simulink model "Pierre_Controller_LTI_2026b"  (R2025b)
settings: Solver=ode1  StartTime=0.0  StopTime=inf  FixedStep=Ts  RelTol=1e-3
PostLoadFcn:
  | , if any(exist('dsrtsu_mdlpostloadfcn', 'file') ~= 0), dsrtsu_mdlpostloadfcn('Execute', bdroot); end,
InitFcn:
  | , if any(exist('rtifpga_mdlclblib', 'file') ~= 0), rtifpga_mdlclblib('Init', bdroot); end,
values from neighbouring files (symbols this model uses):
  BUTTER = ss(A,B,C,D,Ts)    [build_model.m]
  K = opensave.K_final    [build_model.m]
  Px = 1    [build_model.m]
  Py = 1    [build_model.m]
  Pz = 1    [build_model.m]
  S_Sensor = 0.1134    [build_model.m]
  Sen_AX = 2.0176    [build_model.m]
  Sen_AY = 2.011    [build_model.m]
  Sen_AZ = 2.0066    [build_model.m]
  Sen_GX = 0.75481    [build_model.m]
  Sen_GY = 0.75728    [build_model.m]
  Sen_GZ = 0.74931    [build_model.m]
  Sweep_amp = 0.5    [build_model.m]
  Switch_excit = 4    [build_model.m]
  TMS_amp = 2    [build_model.m]
  TMS_freq1 = 80    [build_model.m]
  TMS_freq2 = 0    [build_model.m]
  TMS_freq3 = 0    [build_model.m]
  Ts = 1/Fs    (= 0.001)    [build_model.m]
  V_sat = 2/10    (= 0.2)    [build_model.m]
  V_sat_TMS = 5    [build_model.m]
undefined symbols (not defined in the file or in its folder): R, S
libraries: dspfdesign x15, rti1202lib_adc_class1 x10, rti1202lib_dac_class1 x7, rti1202lib_adc_class2 x6, dspxfrm3 x3, cstblocks x1, simulink x1
(part 2 of 3)

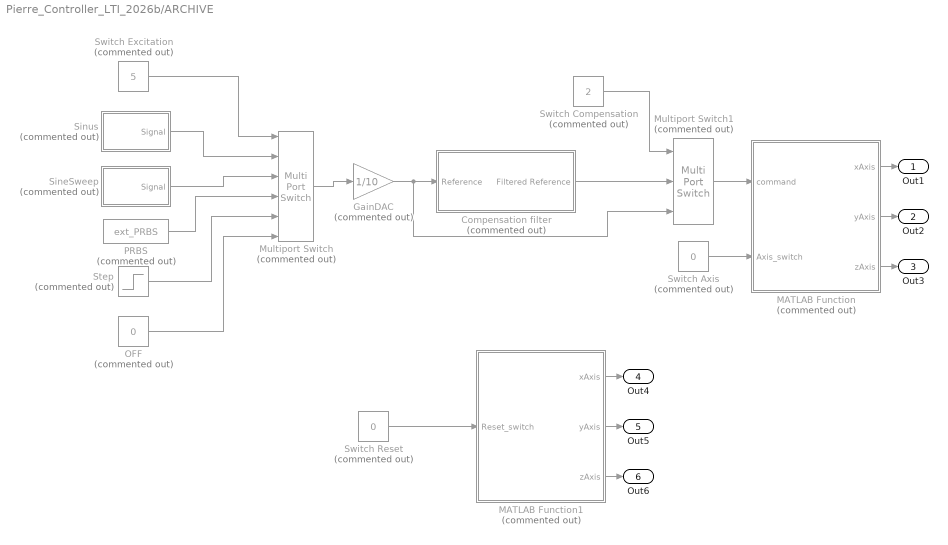
== system Pierre_Controller_LTI_2026b/ARCHIVE ==
  Compensation filter : Subsystem  Commented=on
  GainDAC : Gain  Commented=on  Gain=1/10
  MATLAB Function : MATLAB Function  Commented=on  TreatAsAtomicUnit=on
  MATLAB Function1 : MATLAB Function  Commented=on  TreatAsAtomicUnit=on  SystemSampleTime=Ts
  Multiport Switch : MultiPortSwitch  Commented=on  Inputs=5  DiagnosticForDefault=Warning  SaturateOnIntegerOverflow=off  InputSameDT=off
  Multiport Switch1 : MultiPortSwitch  Commented=on  Inputs=2  DiagnosticForDefault=Warning  SaturateOnIntegerOverflow=off  InputSameDT=off
  OFF : Constant  Commented=on  Value=0
  PRBS : FromWorkspace  Commented=on  VariableName=ext_PRBS  SampleTime=-1
  SineSweep : Subsystem  Commented=on
  Sinus : Subsystem  Commented=on
  Step : Step  Commented=on  Time=5  After=0.5  SampleTime=Ts
  Switch Axis : Constant  Commented=on  Value=0
  Switch Compensation : Constant  Commented=on  Value=2
  Switch Excitation : Constant  Commented=on  Value=5
  Switch Reset : Constant  Commented=on  Value=0  SampleTime=Ts
  Out1 : Outport  VectorParamsAs1DForOutWhenUnconnected=off
  Out2 : Outport  Port=2  VectorParamsAs1DForOutWhenUnconnected=off
  Out3 : Outport  Port=3  VectorParamsAs1DForOutWhenUnconnected=off
  Out4 : Outport  Port=4  VectorParamsAs1DForOutWhenUnconnected=off
  Out5 : Outport  Port=5  VectorParamsAs1DForOutWhenUnconnected=off
  Out6 : Outport  Port=6  VectorParamsAs1DForOutWhenUnconnected=off
  wires:
  PRBS/1 -> Multiport Switch/4
  Switch Axis/1 -> MATLAB Function/2(Axis_switch)
  SineSweep/1(Signal) -> Multiport Switch/3
  Multiport Switch/1 -> GainDAC/1
  Sinus/1(Signal) -> Multiport Switch/2
  Switch Excitation/1 -> Multiport Switch/1
  Switch Compensation/1 -> Multiport Switch1/1
  GainDAC/1 -> Multiport Switch1/3, Compensation filter/1(Reference)
  Compensation filter/1(Filtered Reference) -> Multiport Switch1/2
  OFF/1 -> Multiport Switch/6
  Multiport Switch1/1 -> MATLAB Function/1(command)
  Step/1 -> Multiport Switch/5
  Switch Reset/1 -> MATLAB Function1/1(Reset_switch)
  MATLAB Function1/2(yAxis) -> Out5/1
  MATLAB Function/2(yAxis) -> Out2/1
  MATLAB Function1/1(xAxis) -> Out4/1
  MATLAB Function1/3(zAxis) -> Out6/1
  MATLAB Function/1(xAxis) -> Out1/1
  MATLAB Function/3(zAxis) -> Out3/1

== system Pierre_Controller_LTI_2026b/Clock ==
  Clock : Clock
  Timestamp : Outport  VectorParamsAs1DForOutWhenUnconnected=off
  wires:
  Clock/1 -> Timestamp/1

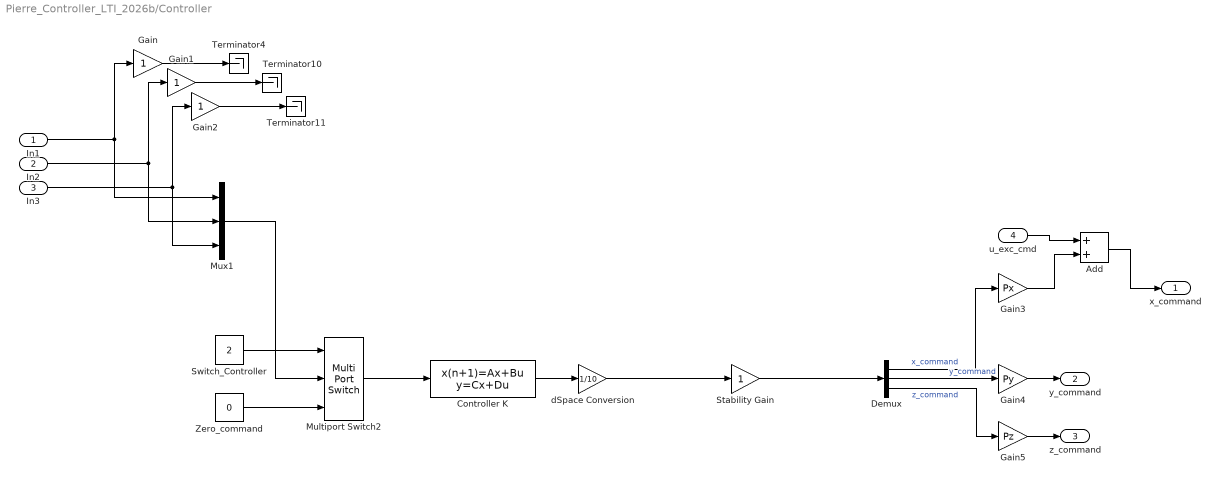
== system Pierre_Controller_LTI_2026b/Controller ==
  In1 : Inport
  In2 : Inport  Port=2
  In3 : Inport  Port=3
  u_exc_cmd : Inport  Port=4
  Add : Sum
  Controller K : DiscreteStateSpace  A=K.A  B=K.B  C=K.C  D=K.D  SampleTime=-1
  Demux : Demux  Outputs=3
  Gain : Gain
  Gain1 : Gain
  Gain2 : Gain
  Gain3 : Gain  Gain=Px
  Gain4 : Gain  Gain=Py
  Gain5 : Gain  Gain=Pz
  Multiport Switch2 : MultiPortSwitch  Inputs=2  DiagnosticForDefault=None  SaturateOnIntegerOverflow=off  InputSameDT=off
  Mux1 : Mux  Inputs=3
  Stability Gain : Gain
  Switch_Controller : Constant  Value=2
  Terminator10 : Terminator
  Terminator11 : Terminator
  Terminator4 : Terminator
  Zero_command : Constant  Value=0  VectorParams1D=off
  dSpace Conversion : Gain  Gain=1/10
  x_command : Outport  VectorParamsAs1DForOutWhenUnconnected=off
  y_command : Outport  Port=2  VectorParamsAs1DForOutWhenUnconnected=off
  z_command : Outport  Port=3  VectorParamsAs1DForOutWhenUnconnected=off
  wires:
  Switch_Controller/1 -> Multiport Switch2/1
  Mux1/1 -> Multiport Switch2/2
  Zero_command/1 -> Multiport Switch2/3
  Demux/2 -> Gain4/1  "y_command"
  Demux/3 -> Gain5/1  "z_command"
  Demux/1 -> Gain3/1  "x_command"
  In2/1 -> Mux1/2, Gain1/1
  In1/1 -> Mux1/1, Gain/1
  In3/1 -> Mux1/3, Gain2/1
  Gain2/1 -> Terminator11/1
  Gain1/1 -> Terminator10/1
  Gain/1 -> Terminator4/1
  Controller K/1 -> dSpace Conversion/1
  dSpace Conversion/1 -> Stability Gain/1
  Multiport Switch2/1 -> Controller K/1
  Gain3/1 -> Add/2
  Gain4/1 -> y_command/1
  Gain5/1 -> z_command/1
  Stability Gain/1 -> Demux/1
  Add/1 -> x_command/1
  u_exc_cmd/1 -> Add/1

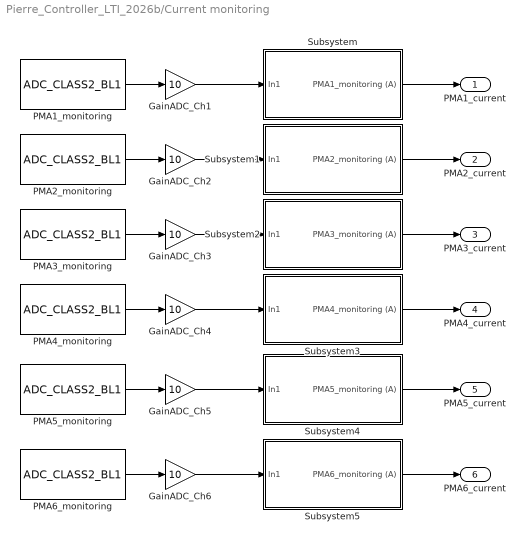
== system Pierre_Controller_LTI_2026b/Current monitoring ==
  GainADC_Ch{1..6} (6 alike) : Gain  Gain=10
  PMA1_monitoring : rti1202lib_adc_class2/ADC_CLASS2_BL1  DSProperties=struct('RTI',struct('Version',uint32(1),'BlockType',struct('isSLSource',uint8(1),'isSLSink',uint8(1),'isHWSource',uint8(0),'isHWSink',uint8(1),'isSetup',uint8(0),'isInline',uint8(1),'isNonInline',uint8(0),'isInterrupt',uint8(0),'isChannelwise',uint8(1)),'IOBoardType',{{'DS120X','STD','ADCC2'}},'UnitType','ADC','Identifier','ADC','DialogType','ML','BlockSet','NONE','SlaveProcessor','NONE'))  RTIBlockInterface=struct('OutputPortsActive',1,'OutputPortsWidth',int32(1),'OutputPortsDataType',{{'SS_DOUBLE'}},'OutputPortsName',{{'ADC'}},'DialogFcn','rti120xstdadcc2adcgui','InitLevel',3,'IconTransparency','on','BlockDisplay',{{['ADC CL2\nChannel: 1'],'center'}},'BlockName',struct('Token',{{'ADC_CLASS2_BL1'}}))  RTIBlockParameters=struct('ChannelNo',{{1,'OFF',[]}},'TLCFileName',{{'rti120xadc_c2_adc','OFF',[]}})  RTISFcnParameters=struct('ChannelNo','int16','TLCFileName','char')  RTIBlockParaDefault=struct('ChannelNo',1,'TLCFileName','rti120xadc_c2_adc')
  PMA2_monitoring : rti1202lib_adc_class2/ADC_CLASS2_BL1  DSProperties=struct('RTI',struct('Version',uint32(1),'BlockType',struct('isSLSource',uint8(1),'isSLSink',uint8(1),'isHWSource',uint8(0),'isHWSink',uint8(1),'isSetup',uint8(0),'isInline',uint8(1),'isNonInline',uint8(0),'isInterrupt',uint8(0),'isChannelwise',uint8(1)),'IOBoardType',{{'DS120X','STD','ADCC2'}},'UnitType','ADC','Identifier','ADC','DialogType','ML','BlockSet','NONE','SlaveProcessor','NONE'))  RTIBlockInterface=struct('OutputPortsActive',1,'OutputPortsWidth',int32(1),'OutputPortsDataType',{{'SS_DOUBLE'}},'OutputPortsName',{{'ADC'}},'DialogFcn','rti120xstdadcc2adcgui','InitLevel',3,'IconTransparency','on','BlockDisplay',{{['ADC CL2\nChannel: 2'],'center'}},'BlockName',struct('Token',{{'ADC_CLASS2_BL1'}}))  RTIBlockParameters=struct('ChannelNo',{{2,'OFF',[]}},'TLCFileName',{{'rti120xadc_c2_adc','OFF',[]}})  RTISFcnParameters=struct('ChannelNo','int16','TLCFileName','char')  RTIBlockParaDefault=struct('ChannelNo',1,'TLCFileName','rti120xadc_c2_adc')
  PMA3_monitoring : rti1202lib_adc_class2/ADC_CLASS2_BL1  DSProperties=struct('RTI',struct('Version',uint32(1),'BlockType',struct('isSLSource',uint8(1),'isSLSink',uint8(1),'isHWSource',uint8(0),'isHWSink',uint8(1),'isSetup',uint8(0),'isInline',uint8(1),'isNonInline',uint8(0),'isInterrupt',uint8(0),'isChannelwise',uint8(1)),'IOBoardType',{{'DS120X','STD','ADCC2'}},'UnitType','ADC','Identifier','ADC','DialogType','ML','BlockSet','NONE','SlaveProcessor','NONE'))  RTIBlockInterface=struct('OutputPortsActive',1,'OutputPortsWidth',int32(1),'OutputPortsDataType',{{'SS_DOUBLE'}},'OutputPortsName',{{'ADC'}},'DialogFcn','rti120xstdadcc2adcgui','InitLevel',3,'IconTransparency','on','BlockDisplay',{{['ADC CL2\nChannel: 3'],'center'}},'BlockName',struct('Token',{{'ADC_CLASS2_BL1'}}))  RTIBlockParameters=struct('ChannelNo',{{3,'OFF',[]}},'TLCFileName',{{'rti120xadc_c2_adc','OFF',[]}})  RTISFcnParameters=struct('ChannelNo','int16','TLCFileName','char')  RTIBlockParaDefault=struct('ChannelNo',1,'TLCFileName','rti120xadc_c2_adc')
  PMA4_monitoring : rti1202lib_adc_class2/ADC_CLASS2_BL1  DSProperties=struct('RTI',struct('Version',uint32(1),'BlockType',struct('isSLSource',uint8(1),'isSLSink',uint8(1),'isHWSource',uint8(0),'isHWSink',uint8(1),'isSetup',uint8(0),'isInline',uint8(1),'isNonInline',uint8(0),'isInterrupt',uint8(0),'isChannelwise',uint8(1)),'IOBoardType',{{'DS120X','STD','ADCC2'}},'UnitType','ADC','Identifier','ADC','DialogType','ML','BlockSet','NONE','SlaveProcessor','NONE'))  RTIBlockInterface=struct('OutputPortsActive',1,'OutputPortsWidth',int32(1),'OutputPortsDataType',{{'SS_DOUBLE'}},'OutputPortsName',{{'ADC'}},'DialogFcn','rti120xstdadcc2adcgui','InitLevel',3,'IconTransparency','on','BlockDisplay',{{['ADC CL2\nChannel: 4'],'center'}},'BlockName',struct('Token',{{'ADC_CLASS2_BL1'}}))  RTIBlockParameters=struct('ChannelNo',{{4,'OFF',[]}},'TLCFileName',{{'rti120xadc_c2_adc','OFF',[]}})  RTISFcnParameters=struct('ChannelNo','int16','TLCFileName','char')  RTIBlockParaDefault=struct('ChannelNo',1,'TLCFileName','rti120xadc_c2_adc')
  PMA5_monitoring : rti1202lib_adc_class2/ADC_CLASS2_BL1  DSProperties=struct('RTI',struct('Version',uint32(1),'BlockType',struct('isSLSource',uint8(1),'isSLSink',uint8(1),'isHWSource',uint8(0),'isHWSink',uint8(1),'isSetup',uint8(0),'isInline',uint8(1),'isNonInline',uint8(0),'isInterrupt',uint8(0),'isChannelwise',uint8(1)),'IOBoardType',{{'DS120X','STD','ADCC2'}},'UnitType','ADC','Identifier','ADC','DialogType','ML','BlockSet','NONE','SlaveProcessor','NONE'))  RTIBlockInterface=struct('OutputPortsActive',1,'OutputPortsWidth',int32(1),'OutputPortsDataType',{{'SS_DOUBLE'}},'OutputPortsName',{{'ADC'}},'DialogFcn','rti120xstdadcc2adcgui','InitLevel',3,'IconTransparency','on','BlockDisplay',{{['ADC CL2\nChannel: 5'],'center'}},'BlockName',struct('Token',{{'ADC_CLASS2_BL1'}}))  RTIBlockParameters=struct('ChannelNo',{{5,'OFF',[]}},'TLCFileName',{{'rti120xadc_c2_adc','OFF',[]}})  RTISFcnParameters=struct('ChannelNo','int16','TLCFileName','char')  RTIBlockParaDefault=struct('ChannelNo',1,'TLCFileName','rti120xadc_c2_adc')
  PMA6_monitoring : rti1202lib_adc_class2/ADC_CLASS2_BL1  DSProperties=struct('RTI',struct('Version',uint32(1),'BlockType',struct('isSLSource',uint8(1),'isSLSink',uint8(1),'isHWSource',uint8(0),'isHWSink',uint8(1),'isSetup',uint8(0),'isInline',uint8(1),'isNonInline',uint8(0),'isInterrupt',uint8(0),'isChannelwise',uint8(1)),'IOBoardType',{{'DS120X','STD','ADCC2'}},'UnitType','ADC','Identifier','ADC','DialogType','ML','BlockSet','NONE','SlaveProcessor','NONE'))  RTIBlockInterface=struct('OutputPortsActive',1,'OutputPortsWidth',int32(1),'OutputPortsDataType',{{'SS_DOUBLE'}},'OutputPortsName',{{'ADC'}},'DialogFcn','rti120xstdadcc2adcgui','InitLevel',3,'IconTransparency','on','BlockDisplay',{{['ADC CL2\nChannel: 6'],'center'}},'BlockName',struct('Token',{{'ADC_CLASS2_BL1'}}))  RTIBlockParameters=struct('ChannelNo',{{6,'OFF',[]}},'TLCFileName',{{'rti120xadc_c2_adc','OFF',[]}})  RTISFcnParameters=struct('ChannelNo','int16','TLCFileName','char')  RTIBlockParaDefault=struct('ChannelNo',1,'TLCFileName','rti120xadc_c2_adc')
  Subsystem : Subsystem
  Subsystem1 : Subsystem
  Subsystem2 : Subsystem
  Subsystem3 : Subsystem
  Subsystem4 : Subsystem
  Subsystem5 : Subsystem
  PMA1_current : Outport  VectorParamsAs1DForOutWhenUnconnected=off
  PMA2_current : Outport  Port=2  VectorParamsAs1DForOutWhenUnconnected=off
  PMA3_current : Outport  Port=3  VectorParamsAs1DForOutWhenUnconnected=off
  PMA4_current : Outport  Port=4  VectorParamsAs1DForOutWhenUnconnected=off
  PMA5_current : Outport  Port=5  VectorParamsAs1DForOutWhenUnconnected=off
  PMA6_current : Outport  Port=6  VectorParamsAs1DForOutWhenUnconnected=off
  wires:
  GainADC_Ch6/1 -> Subsystem5/1(In1)
  PMA5_monitoring/1 -> GainADC_Ch5/1
  PMA6_monitoring/1 -> GainADC_Ch6/1
  GainADC_Ch5/1 -> Subsystem4/1(In1)
  GainADC_Ch1/1 -> Subsystem/1(In1)
  PMA1_monitoring/1 -> GainADC_Ch1/1
  PMA2_monitoring/1 -> GainADC_Ch2/1
  GainADC_Ch2/1 -> Subsystem1/1(In1)
  PMA3_monitoring/1 -> GainADC_Ch3/1
  GainADC_Ch3/1 -> Subsystem2/1(In1)
  GainADC_Ch4/1 -> Subsystem3/1(In1)
  PMA4_monitoring/1 -> GainADC_Ch4/1
  Subsystem/1(PMA1_monitoring (A)) -> PMA1_current/1
  Subsystem1/1(PMA2_monitoring (A)) -> PMA2_current/1
  Subsystem2/1(PMA3_monitoring (A)) -> PMA3_current/1
  Subsystem3/1(PMA4_monitoring (A)) -> PMA4_current/1
  Subsystem4/1(PMA5_monitoring (A)) -> PMA5_current/1
  Subsystem5/1(PMA6_monitoring (A)) -> PMA6_current/1

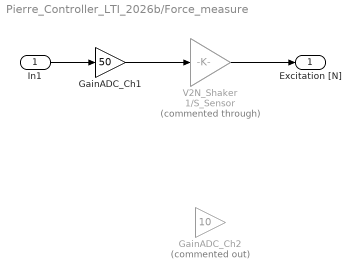
== system Pierre_Controller_LTI_2026b/Force_measure ==
  In1 : Inport
  GainADC_Ch1 : Gain  Gain=50
  GainADC_Ch2 : Gain  Commented=on  Gain=10
  V2N_Shaker : Gain  Commented=through  Gain=1/S_Sensor
  Excitation [N] : Outport  VectorParamsAs1DForOutWhenUnconnected=off
  wires:
  In1/1 -> GainADC_Ch1/1
  V2N_Shaker/1 -> Excitation [N]/1
  GainADC_Ch1/1 -> V2N_Shaker/1

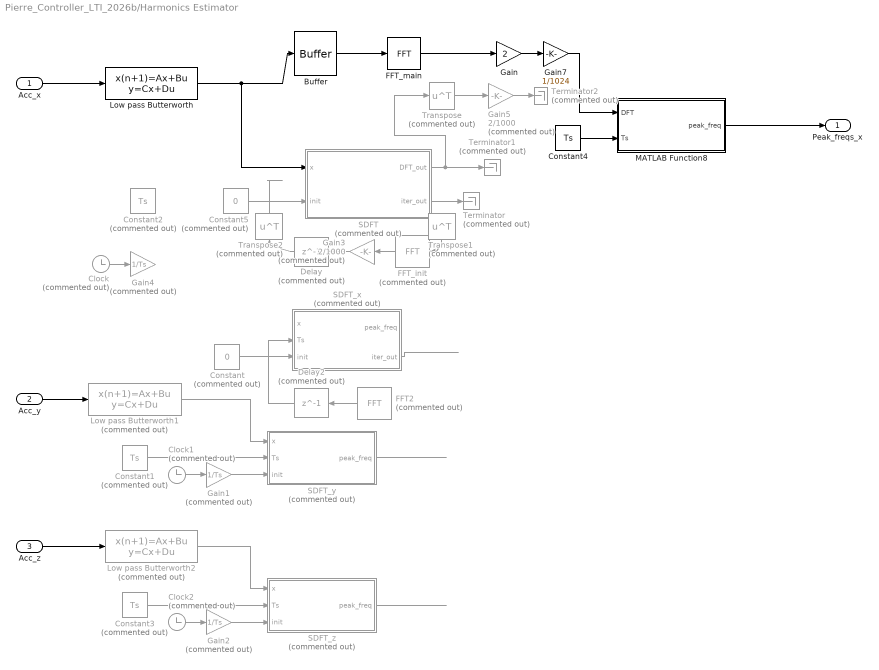
== system Pierre_Controller_LTI_2026b/Harmonics Estimator ==
  Acc_x : Inport
  Acc_y : Inport  Port=2
  Acc_z : Inport  Port=3
  Buffer : Buffer  N=1024  OutputFrames=off
  Clock : Clock  Commented=on
  Clock1 : Clock  Commented=on
  Clock2 : Clock  Commented=on
  Constant : Constant  Commented=on  Value=0
  Constant1 : Constant  Commented=on  Value=Ts  SampleTime=-1
  Constant2 : Constant  Commented=on  Value=Ts  SampleTime=-1
  Constant3 : Constant  Commented=on  Value=Ts  SampleTime=-1
  Constant4 : Constant  Value=Ts  SampleTime=-1
  Constant5 : Constant  Commented=on  Value=0  SampleTime=-1
  Delay : Delay  Commented=on  DelayLength=1  InitialCondition=0
  Delay2 : Delay  Commented=on  DelayLength=1  InitialCondition=0
  FFT2 : dspxfrm3/FFT  Commented=on  FFTImplementation=Auto  CompMethod=Table lookup  TableOpt=NEW  TableOptActive=Speed  BitRevOrder=off  Normalize=off  InheritFFTLength=on  FFTLength=64  WrapInput=on  roundingMode=Floor  overflowMode=off  firstCoeffDataTypeStr=Inherit: Same word length as input  firstCoeffLastDataTypeStr=Inherit: Same word length as input  outputMin=[]  outputMax=[]
  FFT_init : dspxfrm3/FFT  Commented=on  FFTImplementation=Auto  CompMethod=Table lookup  TableOpt=NEW  TableOptActive=Speed  BitRevOrder=off  Normalize=off  InheritFFTLength=on  FFTLength=64  WrapInput=on  roundingMode=Floor  overflowMode=off  firstCoeffDataTypeStr=Inherit: Same word length as input  firstCoeffLastDataTypeStr=Inherit: Same word length as input  outputMin=[]  outputMax=[]
  FFT_main : dspxfrm3/FFT  FFTImplementation=Auto  CompMethod=Table lookup  TableOpt=NEW  TableOptActive=Speed  BitRevOrder=off  Normalize=off  InheritFFTLength=on  FFTLength=64  WrapInput=on  roundingMode=Floor  overflowMode=off  firstCoeffDataTypeStr=Inherit: Same word length as input  firstCoeffLastDataTypeStr=Inherit: Same word length as input  outputMin=[]  outputMax=[]
  Gain : Gain  Gain=2
  Gain1 : Gain  Commented=on  Gain=1/Ts
  Gain2 : Gain  Commented=on  Gain=1/Ts
  Gain3 : Gain  Commented=on  Gain=2/1000
  Gain4 : Gain  Commented=on  Gain=1/Ts
  Gain5 : Gain  Commented=on  Gain=2/1000
  Gain7 : Gain  Gain=1/1024
  Low pass Butterworth : DiscreteStateSpace  A=BUTTER.A  B=BUTTER.B  C=BUTTER.C  D=BUTTER.D  SampleTime=-1
  Low pass Butterworth1 : DiscreteStateSpace  Commented=on  A=BUTTER.A  B=BUTTER.B  C=BUTTER.C  D=BUTTER.D  SampleTime=-1
  Low pass Butterworth2 : DiscreteStateSpace  Commented=on  A=BUTTER.A  B=BUTTER.B  C=BUTTER.C  D=BUTTER.D  SampleTime=-1
  MATLAB Function8 : MATLAB Function  TreatAsAtomicUnit=on
  SDFT : MATLAB Function  Commented=on  TreatAsAtomicUnit=on
  SDFT_x : MATLAB Function  Commented=on  TreatAsAtomicUnit=on
  SDFT_y : MATLAB Function  Commented=on  TreatAsAtomicUnit=on
  SDFT_z : MATLAB Function  Commented=on  TreatAsAtomicUnit=on
  Terminator : Terminator  Commented=on
  Terminator1 : Terminator  Commented=on
  Terminator2 : Terminator  Commented=on
  Transpose : Math  Commented=on  Operator=transpose
  Transpose1 : Math  Commented=on  Operator=transpose
  Transpose2 : Math  Commented=on  Operator=transpose
  Peak_freqs_x : Outport  VectorParamsAs1DForOutWhenUnconnected=off
  wires:
  Clock/1 -> Gain4/1
  Acc_x/1 -> Low pass Butterworth/1
  Constant1/1 -> SDFT_y/2(Ts)
  Clock1/1 -> Gain1/1
  Gain1/1 -> SDFT_y/3(init)
  SDFT_y/1(peak_freq) -> ?
  Low pass Butterworth1/1 -> SDFT_y/1(x)
  Acc_y/1 -> Low pass Butterworth1/1
  Constant3/1 -> SDFT_z/2(Ts)
  Clock2/1 -> Gain2/1
  Gain2/1 -> SDFT_z/3(init)
  SDFT_z/1(peak_freq) -> ?
  Low pass Butterworth2/1 -> SDFT_z/1(x)
  Acc_z/1 -> Low pass Butterworth2/1
  SDFT_x/2(iter_out) -> ?
  Buffer/1 -> FFT_main/1
  Gain/1 -> Gain7/1
  FFT_main/1 -> Gain/1
  Constant4/1 -> MATLAB Function8/2(Ts)
  MATLAB Function8/1(peak_freq) -> Peak_freqs_x/1
  Constant/1 -> SDFT_x/3(init)
  Low pass Butterworth/1 -> SDFT/1(x), Buffer/1
  FFT_init/1 -> Gain3/1
  FFT2/1 -> Delay2/1
  ? -> FFT2/1
  Delay2/1 -> SDFT_x/2(Ts)
  Constant5/1 -> SDFT/2(init)
  SDFT/2(iter_out) -> Terminator/1
  Delay/1 -> Transpose2/1
  SDFT/1(DFT_out) -> Transpose/1, Terminator1/1
  Transpose1/1 -> FFT_init/1
  Transpose2/1 -> ?
  Gain3/1 -> Delay/1
  Transpose/1 -> Gain5/1
  Gain7/1 -> MATLAB Function8/1(DFT)
  Gain5/1 -> Terminator2/1

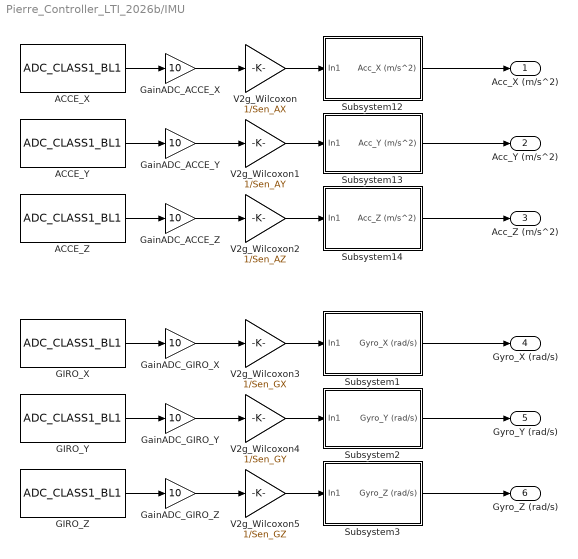
== system Pierre_Controller_LTI_2026b/IMU ==
  ACCE_X : rti1202lib_adc_class1/ADC_CLASS1_BL1  DSProperties=struct('RTI',struct('Version',uint32(1),'BlockType',struct('isSLSource',uint8(1),'isSLSink',uint8(1),'isHWSource',uint8(0),'isHWSink',uint8(1),'isSetup',uint8(0),'isInline',uint8(1),'isNonInline',uint8(0),'isInterrupt',uint8(0),'isChannelwise',uint8(1)),'IOBoardType',{{'DS120X','STD','ADCC1'}},'UnitType','ADC','Identifier','ADC','DialogType','ML','BlockSet','NONE','SlaveProcessor','NONE'))  RTIBlockInterface=struct('InputPortsActive',0,'InputPortsWidth',int32(1),'InputPortsDataType',{{'SS_BOOLEAN'}},'InputPortsName',{{'Continue'}},'OutputPortsActive',[1 0],'OutputPortsWidth',int32([1 1]),'OutputPortsDataType',{{'SS_DOUBLE','SS_INT16'}},'OutputPortsName',{{'ADC','Status'}},'DialogFcn','rti120xstdadcc1adcgui','SampleTime',{{-1}},'InitLevel',3,'IconTransparency','on','BlockDisplay',{{['ADC CL1\nChannel: 9'],'center'}},'BlockName',struct('Token',{{'ADC_CLASS1_BL1'}}))  RTIBlockParameters=struct('ReadMode',{{1,'OFF',[1 2]}},'ChannelNo',{{9,'OFF',[]}},'ConversionMode',{{1,'OFF',[1 2]}},'TriggerSource',{{1,'OFF',[1 2]}},'TriggerLineIn',{{1,'OFF',[1 16]}},'SampleMode',{{1,'OFF',[1 2]}},'BurstTriggerSource',{{1,'OFF',[1 2]}},'BurstTriggerLine',{{1,'OFF',[1 16]}},'ConvTriggerSource',{{3,'OFF',[1 3]}},'ConvTriggerLine',{{1,'OFF',[1 16]}},'ConvPeriod',{{'100e-6','OFF',[1e-6 1.34]}},'ConvPeriodCheck',{{0,'OFF',[]}},'BurstSize',{{'10','OFF',[]}},'BurstSizeCheck',{{0,'OFF',[]}},'DataSetOffset',{{'0','OFF',[]}},'DataSetOffsetCheck',{{0,'OFF',[]}},'DataSetLength',{{'1','OFF',[]}},'DataSetLengthCheck',{{0,'OFF',[]}},'EnableTriggerEvent',{{0,'OFF',[0 1]}},'TriggerMode',{{2,'OFF',[1 3]}},'TriggerLineOut',{{1,'OFF',[1 16]}},'ADCSWStartEnable',{{0,'OFF',[0 1]}},'SampleTime',{{'-1','OFF',[-1 inf]}},'SampleTimeCheck',{{1,'OFF',[]}},'StatusPortEnable',{{0,'OFF',[0 1]}},'TLCFileName',{{'rti120xadc_c1_adc','OFF',[]}})  RTISFcnParameters=struct('ReadMode','int16','ChannelNo','int16','ConversionMode','int16','TriggerSource','int16','TriggerLineIn','int16','SampleMode','int16','BurstTriggerSource','int16','BurstTriggerLine','int16','ConvTriggerSource','int16','ConvTriggerLine','int16','ConvPeriod','double','BurstSize','int16','DataSetOffset','int16','DataSetLength','int16','EnableTriggerEvent','int16','TriggerMode','int16','TriggerLineOut','int16','ADCSWStartEnable','int16','SampleTime','double','StatusPortEnable','int16','TLCFileName','char')  RTIBlockParaDefault=struct('ReadMode',1,'ChannelNo',1,'ConversionMode',1,'TriggerSource',1,'TriggerLineIn',1,'SampleMode',1,'BurstTriggerSource',1,'BurstTriggerLine',1,'ConvTriggerSource',3,'ConvTriggerLine',1,'ConvPeriod',0.0001,'ConvPeriodCheck',0,'BurstSize',10,'BurstSizeCheck',0,'DataSetOffset',0,'DataSetOffsetCheck',0,'DataSetLength',1,'DataSetLengthCheck',0,'EnableTriggerEvent',0,'TriggerMode',2,'TriggerLineOut',1,'ADCSWStartEnable',0,'SampleTime',-1,'SampleTimeCheck',1,'StatusPortEnable',0,'TLCFileName','rti120xadc_c1_adc')
  ACCE_Y : rti1202lib_adc_class1/ADC_CLASS1_BL1  DSProperties=struct('RTI',struct('Version',uint32(1),'BlockType',struct('isSLSource',uint8(1),'isSLSink',uint8(1),'isHWSource',uint8(0),'isHWSink',uint8(1),'isSetup',uint8(0),'isInline',uint8(1),'isNonInline',uint8(0),'isInterrupt',uint8(0),'isChannelwise',uint8(1)),'IOBoardType',{{'DS120X','STD','ADCC1'}},'UnitType','ADC','Identifier','ADC','DialogType','ML','BlockSet','NONE','SlaveProcessor','NONE'))  RTIBlockInterface=struct('InputPortsActive',0,'InputPortsWidth',int32(1),'InputPortsDataType',{{'SS_BOOLEAN'}},'InputPortsName',{{'Continue'}},'OutputPortsActive',[1 0],'OutputPortsWidth',int32([1 1]),'OutputPortsDataType',{{'SS_DOUBLE','SS_INT16'}},'OutputPortsName',{{'ADC','Status'}},'DialogFcn','rti120xstdadcc1adcgui','SampleTime',{{-1}},'InitLevel',3,'IconTransparency','on','BlockDisplay',{{['ADC CL1\nChannel: 10'],'center'}},'BlockName',struct('Token',{{'ADC_CLASS1_BL1'}}))  RTIBlockParameters=struct('ReadMode',{{1,'OFF',[1 2]}},'ChannelNo',{{10,'OFF',[]}},'ConversionMode',{{1,'OFF',[1 2]}},'TriggerSource',{{1,'OFF',[1 2]}},'TriggerLineIn',{{1,'OFF',[1 16]}},'SampleMode',{{1,'OFF',[1 2]}},'BurstTriggerSource',{{1,'OFF',[1 2]}},'BurstTriggerLine',{{1,'OFF',[1 16]}},'ConvTriggerSource',{{3,'OFF',[1 3]}},'ConvTriggerLine',{{1,'OFF',[1 16]}},'ConvPeriod',{{'100e-6','OFF',[1e-6 1.34]}},'ConvPeriodCheck',{{0,'OFF',[]}},'BurstSize',{{'10','OFF',[]}},'BurstSizeCheck',{{0,'OFF',[]}},'DataSetOffset',{{'0','OFF',[]}},'DataSetOffsetCheck',{{0,'OFF',[]}},'DataSetLength',{{'1','OFF',[]}},'DataSetLengthCheck',{{0,'OFF',[]}},'EnableTriggerEvent',{{0,'OFF',[0 1]}},'TriggerMode',{{2,'OFF',[1 3]}},'TriggerLineOut',{{1,'OFF',[1 16]}},'ADCSWStartEnable',{{0,'OFF',[0 1]}},'SampleTime',{{'-1','OFF',[-1 inf]}},'SampleTimeCheck',{{1,'OFF',[]}},'StatusPortEnable',{{0,'OFF',[0 1]}},'TLCFileName',{{'rti120xadc_c1_adc','OFF',[]}})  RTISFcnParameters=struct('ReadMode','int16','ChannelNo','int16','ConversionMode','int16','TriggerSource','int16','TriggerLineIn','int16','SampleMode','int16','BurstTriggerSource','int16','BurstTriggerLine','int16','ConvTriggerSource','int16','ConvTriggerLine','int16','ConvPeriod','double','BurstSize','int16','DataSetOffset','int16','DataSetLength','int16','EnableTriggerEvent','int16','TriggerMode','int16','TriggerLineOut','int16','ADCSWStartEnable','int16','SampleTime','double','StatusPortEnable','int16','TLCFileName','char')  RTIBlockParaDefault=struct('ReadMode',1,'ChannelNo',1,'ConversionMode',1,'TriggerSource',1,'TriggerLineIn',1,'SampleMode',1,'BurstTriggerSource',1,'BurstTriggerLine',1,'ConvTriggerSource',3,'ConvTriggerLine',1,'ConvPeriod',0.0001,'ConvPeriodCheck',0,'BurstSize',10,'BurstSizeCheck',0,'DataSetOffset',0,'DataSetOffsetCheck',0,'DataSetLength',1,'DataSetLengthCheck',0,'EnableTriggerEvent',0,'TriggerMode',2,'TriggerLineOut',1,'ADCSWStartEnable',0,'SampleTime',-1,'SampleTimeCheck',1,'StatusPortEnable',0,'TLCFileName','rti120xadc_c1_adc')
  ACCE_Z : rti1202lib_adc_class1/ADC_CLASS1_BL1  DSProperties=struct('RTI',struct('Version',uint32(1),'BlockType',struct('isSLSource',uint8(1),'isSLSink',uint8(1),'isHWSource',uint8(0),'isHWSink',uint8(1),'isSetup',uint8(0),'isInline',uint8(1),'isNonInline',uint8(0),'isInterrupt',uint8(0),'isChannelwise',uint8(1)),'IOBoardType',{{'DS120X','STD','ADCC1'}},'UnitType','ADC','Identifier','ADC','DialogType','ML','BlockSet','NONE','SlaveProcessor','NONE'))  RTIBlockInterface=struct('InputPortsActive',0,'InputPortsWidth',int32(1),'InputPortsDataType',{{'SS_BOOLEAN'}},'InputPortsName',{{'Continue'}},'OutputPortsActive',[1 0],'OutputPortsWidth',int32([1 1]),'OutputPortsDataType',{{'SS_DOUBLE','SS_INT16'}},'OutputPortsName',{{'ADC','Status'}},'DialogFcn','rti120xstdadcc1adcgui','SampleTime',{{-1}},'InitLevel',3,'IconTransparency','on','BlockDisplay',{{['ADC CL1\nChannel: 11'],'center'}},'BlockName',struct('Token',{{'ADC_CLASS1_BL1'}}))  RTIBlockParameters=struct('ReadMode',{{1,'OFF',[1 2]}},'ChannelNo',{{11,'OFF',[]}},'ConversionMode',{{1,'OFF',[1 2]}},'TriggerSource',{{1,'OFF',[1 2]}},'TriggerLineIn',{{1,'OFF',[1 16]}},'SampleMode',{{1,'OFF',[1 2]}},'BurstTriggerSource',{{1,'OFF',[1 2]}},'BurstTriggerLine',{{1,'OFF',[1 16]}},'ConvTriggerSource',{{3,'OFF',[1 3]}},'ConvTriggerLine',{{1,'OFF',[1 16]}},'ConvPeriod',{{'100e-6','OFF',[1e-6 1.34]}},'ConvPeriodCheck',{{0,'OFF',[]}},'BurstSize',{{'10','OFF',[]}},'BurstSizeCheck',{{0,'OFF',[]}},'DataSetOffset',{{'0','OFF',[]}},'DataSetOffsetCheck',{{0,'OFF',[]}},'DataSetLength',{{'1','OFF',[]}},'DataSetLengthCheck',{{0,'OFF',[]}},'EnableTriggerEvent',{{0,'OFF',[0 1]}},'TriggerMode',{{2,'OFF',[1 3]}},'TriggerLineOut',{{1,'OFF',[1 16]}},'ADCSWStartEnable',{{0,'OFF',[0 1]}},'SampleTime',{{'-1','OFF',[-1 inf]}},'SampleTimeCheck',{{1,'OFF',[]}},'StatusPortEnable',{{0,'OFF',[0 1]}},'TLCFileName',{{'rti120xadc_c1_adc','OFF',[]}})  RTISFcnParameters=struct('ReadMode','int16','ChannelNo','int16','ConversionMode','int16','TriggerSource','int16','TriggerLineIn','int16','SampleMode','int16','BurstTriggerSource','int16','BurstTriggerLine','int16','ConvTriggerSource','int16','ConvTriggerLine','int16','ConvPeriod','double','BurstSize','int16','DataSetOffset','int16','DataSetLength','int16','EnableTriggerEvent','int16','TriggerMode','int16','TriggerLineOut','int16','ADCSWStartEnable','int16','SampleTime','double','StatusPortEnable','int16','TLCFileName','char')  RTIBlockParaDefault=struct('ReadMode',1,'ChannelNo',1,'ConversionMode',1,'TriggerSource',1,'TriggerLineIn',1,'SampleMode',1,'BurstTriggerSource',1,'BurstTriggerLine',1,'ConvTriggerSource',3,'ConvTriggerLine',1,'ConvPeriod',0.0001,'ConvPeriodCheck',0,'BurstSize',10,'BurstSizeCheck',0,'DataSetOffset',0,'DataSetOffsetCheck',0,'DataSetLength',1,'DataSetLengthCheck',0,'EnableTriggerEvent',0,'TriggerMode',2,'TriggerLineOut',1,'ADCSWStartEnable',0,'SampleTime',-1,'SampleTimeCheck',1,'StatusPortEnable',0,'TLCFileName','rti120xadc_c1_adc')
  GIRO_X : rti1202lib_adc_class1/ADC_CLASS1_BL1  DSProperties=struct('RTI',struct('Version',uint32(1),'BlockType',struct('isSLSource',uint8(1),'isSLSink',uint8(1),'isHWSource',uint8(0),'isHWSink',uint8(1),'isSetup',uint8(0),'isInline',uint8(1),'isNonInline',uint8(0),'isInterrupt',uint8(0),'isChannelwise',uint8(1)),'IOBoardType',{{'DS120X','STD','ADCC1'}},'UnitType','ADC','Identifier','ADC','DialogType','ML','BlockSet','NONE','SlaveProcessor','NONE'))  RTIBlockInterface=struct('InputPortsActive',0,'InputPortsWidth',int32(1),'InputPortsDataType',{{'SS_BOOLEAN'}},'InputPortsName',{{'Continue'}},'OutputPortsActive',[1 0],'OutputPortsWidth',int32([1 1]),'OutputPortsDataType',{{'SS_DOUBLE','SS_INT16'}},'OutputPortsName',{{'ADC','Status'}},'DialogFcn','rti120xstdadcc1adcgui','SampleTime',{{-1}},'InitLevel',3,'IconTransparency','on','BlockDisplay',{{['ADC CL1\nChannel: 17'],'center'}},'BlockName',struct('Token',{{'ADC_CLASS1_BL1'}}))  RTIBlockParameters=struct('ReadMode',{{1,'OFF',[1 2]}},'ChannelNo',{{17,'OFF',[]}},'ConversionMode',{{1,'OFF',[1 2]}},'TriggerSource',{{1,'OFF',[1 2]}},'TriggerLineIn',{{1,'OFF',[1 16]}},'SampleMode',{{1,'OFF',[1 2]}},'BurstTriggerSource',{{1,'OFF',[1 2]}},'BurstTriggerLine',{{1,'OFF',[1 16]}},'ConvTriggerSource',{{3,'OFF',[1 3]}},'ConvTriggerLine',{{1,'OFF',[1 16]}},'ConvPeriod',{{'100e-6','OFF',[1e-6 1.34]}},'ConvPeriodCheck',{{0,'OFF',[]}},'BurstSize',{{'10','OFF',[]}},'BurstSizeCheck',{{0,'OFF',[]}},'DataSetOffset',{{'0','OFF',[]}},'DataSetOffsetCheck',{{0,'OFF',[]}},'DataSetLength',{{'1','OFF',[]}},'DataSetLengthCheck',{{0,'OFF',[]}},'EnableTriggerEvent',{{0,'OFF',[0 1]}},'TriggerMode',{{2,'OFF',[1 3]}},'TriggerLineOut',{{1,'OFF',[1 16]}},'ADCSWStartEnable',{{0,'OFF',[0 1]}},'SampleTime',{{'-1','OFF',[-1 inf]}},'SampleTimeCheck',{{1,'OFF',[]}},'StatusPortEnable',{{0,'OFF',[0 1]}},'TLCFileName',{{'rti120xadc_c1_adc','OFF',[]}})  RTISFcnParameters=struct('ReadMode','int16','ChannelNo','int16','ConversionMode','int16','TriggerSource','int16','TriggerLineIn','int16','SampleMode','int16','BurstTriggerSource','int16','BurstTriggerLine','int16','ConvTriggerSource','int16','ConvTriggerLine','int16','ConvPeriod','double','BurstSize','int16','DataSetOffset','int16','DataSetLength','int16','EnableTriggerEvent','int16','TriggerMode','int16','TriggerLineOut','int16','ADCSWStartEnable','int16','SampleTime','double','StatusPortEnable','int16','TLCFileName','char')  RTIBlockParaDefault=struct('ReadMode',1,'ChannelNo',1,'ConversionMode',1,'TriggerSource',1,'TriggerLineIn',1,'SampleMode',1,'BurstTriggerSource',1,'BurstTriggerLine',1,'ConvTriggerSource',3,'ConvTriggerLine',1,'ConvPeriod',0.0001,'ConvPeriodCheck',0,'BurstSize',10,'BurstSizeCheck',0,'DataSetOffset',0,'DataSetOffsetCheck',0,'DataSetLength',1,'DataSetLengthCheck',0,'EnableTriggerEvent',0,'TriggerMode',2,'TriggerLineOut',1,'ADCSWStartEnable',0,'SampleTime',-1,'SampleTimeCheck',1,'StatusPortEnable',0,'TLCFileName','rti120xadc_c1_adc')
  GIRO_Y : rti1202lib_adc_class1/ADC_CLASS1_BL1  DSProperties=struct('RTI',struct('Version',uint32(1),'BlockType',struct('isSLSource',uint8(1),'isSLSink',uint8(1),'isHWSource',uint8(0),'isHWSink',uint8(1),'isSetup',uint8(0),'isInline',uint8(1),'isNonInline',uint8(0),'isInterrupt',uint8(0),'isChannelwise',uint8(1)),'IOBoardType',{{'DS120X','STD','ADCC1'}},'UnitType','ADC','Identifier','ADC','DialogType','ML','BlockSet','NONE','SlaveProcessor','NONE'))  RTIBlockInterface=struct('InputPortsActive',0,'InputPortsWidth',int32(1),'InputPortsDataType',{{'SS_BOOLEAN'}},'InputPortsName',{{'Continue'}},'OutputPortsActive',[1 0],'OutputPortsWidth',int32([1 1]),'OutputPortsDataType',{{'SS_DOUBLE','SS_INT16'}},'OutputPortsName',{{'ADC','Status'}},'DialogFcn','rti120xstdadcc1adcgui','SampleTime',{{-1}},'InitLevel',3,'IconTransparency','on','BlockDisplay',{{['ADC CL1\nChannel: 18'],'center'}},'BlockName',struct('Token',{{'ADC_CLASS1_BL1'}}))  RTIBlockParameters=struct('ReadMode',{{1,'OFF',[1 2]}},'ChannelNo',{{18,'OFF',[]}},'ConversionMode',{{1,'OFF',[1 2]}},'TriggerSource',{{1,'OFF',[1 2]}},'TriggerLineIn',{{1,'OFF',[1 16]}},'SampleMode',{{1,'OFF',[1 2]}},'BurstTriggerSource',{{1,'OFF',[1 2]}},'BurstTriggerLine',{{1,'OFF',[1 16]}},'ConvTriggerSource',{{3,'OFF',[1 3]}},'ConvTriggerLine',{{1,'OFF',[1 16]}},'ConvPeriod',{{'100e-6','OFF',[1e-6 1.34]}},'ConvPeriodCheck',{{0,'OFF',[]}},'BurstSize',{{'10','OFF',[]}},'BurstSizeCheck',{{0,'OFF',[]}},'DataSetOffset',{{'0','OFF',[]}},'DataSetOffsetCheck',{{0,'OFF',[]}},'DataSetLength',{{'1','OFF',[]}},'DataSetLengthCheck',{{0,'OFF',[]}},'EnableTriggerEvent',{{0,'OFF',[0 1]}},'TriggerMode',{{2,'OFF',[1 3]}},'TriggerLineOut',{{1,'OFF',[1 16]}},'ADCSWStartEnable',{{0,'OFF',[0 1]}},'SampleTime',{{'-1','OFF',[-1 inf]}},'SampleTimeCheck',{{1,'OFF',[]}},'StatusPortEnable',{{0,'OFF',[0 1]}},'TLCFileName',{{'rti120xadc_c1_adc','OFF',[]}})  RTISFcnParameters=struct('ReadMode','int16','ChannelNo','int16','ConversionMode','int16','TriggerSource','int16','TriggerLineIn','int16','SampleMode','int16','BurstTriggerSource','int16','BurstTriggerLine','int16','ConvTriggerSource','int16','ConvTriggerLine','int16','ConvPeriod','double','BurstSize','int16','DataSetOffset','int16','DataSetLength','int16','EnableTriggerEvent','int16','TriggerMode','int16','TriggerLineOut','int16','ADCSWStartEnable','int16','SampleTime','double','StatusPortEnable','int16','TLCFileName','char')  RTIBlockParaDefault=struct('ReadMode',1,'ChannelNo',1,'ConversionMode',1,'TriggerSource',1,'TriggerLineIn',1,'SampleMode',1,'BurstTriggerSource',1,'BurstTriggerLine',1,'ConvTriggerSource',3,'ConvTriggerLine',1,'ConvPeriod',0.0001,'ConvPeriodCheck',0,'BurstSize',10,'BurstSizeCheck',0,'DataSetOffset',0,'DataSetOffsetCheck',0,'DataSetLength',1,'DataSetLengthCheck',0,'EnableTriggerEvent',0,'TriggerMode',2,'TriggerLineOut',1,'ADCSWStartEnable',0,'SampleTime',-1,'SampleTimeCheck',1,'StatusPortEnable',0,'TLCFileName','rti120xadc_c1_adc')
  GIRO_Z : rti1202lib_adc_class1/ADC_CLASS1_BL1  DSProperties=struct('RTI',struct('Version',uint32(1),'BlockType',struct('isSLSource',uint8(1),'isSLSink',uint8(1),'isHWSource',uint8(0),'isHWSink',uint8(1),'isSetup',uint8(0),'isInline',uint8(1),'isNonInline',uint8(0),'isInterrupt',uint8(0),'isChannelwise',uint8(1)),'IOBoardType',{{'DS120X','STD','ADCC1'}},'UnitType','ADC','Identifier','ADC','DialogType','ML','BlockSet','NONE','SlaveProcessor','NONE'))  RTIBlockInterface=struct('InputPortsActive',0,'InputPortsWidth',int32(1),'InputPortsDataType',{{'SS_BOOLEAN'}},'InputPortsName',{{'Continue'}},'OutputPortsActive',[1 0],'OutputPortsWidth',int32([1 1]),'OutputPortsDataType',{{'SS_DOUBLE','SS_INT16'}},'OutputPortsName',{{'ADC','Status'}},'DialogFcn','rti120xstdadcc1adcgui','SampleTime',{{-1}},'InitLevel',3,'IconTransparency','on','BlockDisplay',{{['ADC CL1\nChannel: 19'],'center'}},'BlockName',struct('Token',{{'ADC_CLASS1_BL1'}}))  RTIBlockParameters=struct('ReadMode',{{1,'OFF',[1 2]}},'ChannelNo',{{19,'OFF',[]}},'ConversionMode',{{1,'OFF',[1 2]}},'TriggerSource',{{1,'OFF',[1 2]}},'TriggerLineIn',{{1,'OFF',[1 16]}},'SampleMode',{{1,'OFF',[1 2]}},'BurstTriggerSource',{{1,'OFF',[1 2]}},'BurstTriggerLine',{{1,'OFF',[1 16]}},'ConvTriggerSource',{{3,'OFF',[1 3]}},'ConvTriggerLine',{{1,'OFF',[1 16]}},'ConvPeriod',{{'100e-6','OFF',[1e-6 1.34]}},'ConvPeriodCheck',{{0,'OFF',[]}},'BurstSize',{{'10','OFF',[]}},'BurstSizeCheck',{{0,'OFF',[]}},'DataSetOffset',{{'0','OFF',[]}},'DataSetOffsetCheck',{{0,'OFF',[]}},'DataSetLength',{{'1','OFF',[]}},'DataSetLengthCheck',{{0,'OFF',[]}},'EnableTriggerEvent',{{0,'OFF',[0 1]}},'TriggerMode',{{2,'OFF',[1 3]}},'TriggerLineOut',{{1,'OFF',[1 16]}},'ADCSWStartEnable',{{0,'OFF',[0 1]}},'SampleTime',{{'-1','OFF',[-1 inf]}},'SampleTimeCheck',{{1,'OFF',[]}},'StatusPortEnable',{{0,'OFF',[0 1]}},'TLCFileName',{{'rti120xadc_c1_adc','OFF',[]}})  RTISFcnParameters=struct('ReadMode','int16','ChannelNo','int16','ConversionMode','int16','TriggerSource','int16','TriggerLineIn','int16','SampleMode','int16','BurstTriggerSource','int16','BurstTriggerLine','int16','ConvTriggerSource','int16','ConvTriggerLine','int16','ConvPeriod','double','BurstSize','int16','DataSetOffset','int16','DataSetLength','int16','EnableTriggerEvent','int16','TriggerMode','int16','TriggerLineOut','int16','ADCSWStartEnable','int16','SampleTime','double','StatusPortEnable','int16','TLCFileName','char')  RTIBlockParaDefault=struct('ReadMode',1,'ChannelNo',1,'ConversionMode',1,'TriggerSource',1,'TriggerLineIn',1,'SampleMode',1,'BurstTriggerSource',1,'BurstTriggerLine',1,'ConvTriggerSource',3,'ConvTriggerLine',1,'ConvPeriod',0.0001,'ConvPeriodCheck',0,'BurstSize',10,'BurstSizeCheck',0,'DataSetOffset',0,'DataSetOffsetCheck',0,'DataSetLength',1,'DataSetLengthCheck',0,'EnableTriggerEvent',0,'TriggerMode',2,'TriggerLineOut',1,'ADCSWStartEnable',0,'SampleTime',-1,'SampleTimeCheck',1,'StatusPortEnable',0,'TLCFileName','rti120xadc_c1_adc')
  GainADC_ACCE_X : Gain  Gain=10
  GainADC_ACCE_Y : Gain  Gain=10
  GainADC_ACCE_Z : Gain  Gain=10
  GainADC_GIRO_X : Gain  Gain=10
  GainADC_GIRO_Y : Gain  Gain=10
  GainADC_GIRO_Z : Gain  Gain=10
  Subsystem1 : Subsystem
  Subsystem12 : Subsystem
  Subsystem13 : Subsystem
  Subsystem14 : Subsystem
  Subsystem2 : Subsystem
  Subsystem3 : Subsystem
  V2g_Wilcoxon : Gain  Gain=1/Sen_AX
  V2g_Wilcoxon1 : Gain  Gain=1/Sen_AY
  V2g_Wilcoxon2 : Gain  Gain=1/Sen_AZ
  V2g_Wilcoxon3 : Gain  Gain=1/Sen_GX
  V2g_Wilcoxon4 : Gain  Gain=1/Sen_GY
  V2g_Wilcoxon5 : Gain  Gain=1/Sen_GZ
  Acc_X (m/s^2) : Outport  VectorParamsAs1DForOutWhenUnconnected=off
  Acc_Y (m/s^2) : Outport  Port=2  VectorParamsAs1DForOutWhenUnconnected=off
  Acc_Z (m/s^2) : Outport  Port=3  VectorParamsAs1DForOutWhenUnconnected=off
  Gyro_X (rad/s) : Outport  Port=4  VectorParamsAs1DForOutWhenUnconnected=off
  Gyro_Y (rad/s) : Outport  Port=5  VectorParamsAs1DForOutWhenUnconnected=off
  Gyro_Z (rad/s) : Outport  Port=6  VectorParamsAs1DForOutWhenUnconnected=off
  wires:
  ACCE_X/1 -> GainADC_ACCE_X/1
  Subsystem2/1(Gyro_Y (rad/s)) -> Gyro_Y (rad/s)/1
  GIRO_Y/1 -> GainADC_GIRO_Y/1
  GainADC_GIRO_Y/1 -> V2g_Wilcoxon4/1
  V2g_Wilcoxon3/1 -> Subsystem1/1(In1)
  GainADC_GIRO_Z/1 -> V2g_Wilcoxon5/1
  V2g_Wilcoxon1/1 -> Subsystem13/1(In1)
  Subsystem13/1(Acc_Y (m/s^2)) -> Acc_Y (m/s^2)/1
  Subsystem1/1(Gyro_X (rad/s)) -> Gyro_X (rad/s)/1
  Subsystem12/1(Acc_X (m/s^2)) -> Acc_X (m/s^2)/1
  GainADC_ACCE_X/1 -> V2g_Wilcoxon/1
  V2g_Wilcoxon2/1 -> Subsystem14/1(In1)
  V2g_Wilcoxon/1 -> Subsystem12/1(In1)
  Subsystem3/1(Gyro_Z (rad/s)) -> Gyro_Z (rad/s)/1
  GIRO_X/1 -> GainADC_GIRO_X/1
  V2g_Wilcoxon4/1 -> Subsystem2/1(In1)
  GainADC_GIRO_X/1 -> V2g_Wilcoxon3/1
  Subsystem14/1(Acc_Z (m/s^2)) -> Acc_Z (m/s^2)/1
  ACCE_Z/1 -> GainADC_ACCE_Z/1
  GIRO_Z/1 -> GainADC_GIRO_Z/1
  GainADC_ACCE_Z/1 -> V2g_Wilcoxon2/1
  GainADC_ACCE_Y/1 -> V2g_Wilcoxon1/1
  ACCE_Y/1 -> GainADC_ACCE_Y/1
  V2g_Wilcoxon5/1 -> Subsystem3/1(In1)

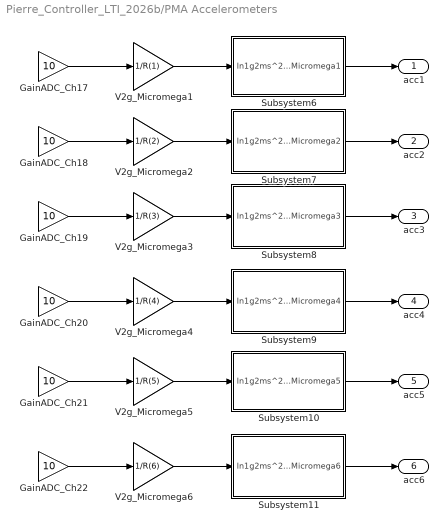
== system Pierre_Controller_LTI_2026b/PMA Accelerometers ==
  GainADC_Ch{17..22} (6 alike) : Gain  Gain=10
  Subsystem10 : Subsystem
  Subsystem11 : Subsystem
  Subsystem6 : Subsystem
  Subsystem7 : Subsystem
  Subsystem8 : Subsystem
  Subsystem9 : Subsystem
  V2g_Micromega1 : Gain  Gain=1/R(1)
  V2g_Micromega2 : Gain  Gain=1/R(2)
  V2g_Micromega3 : Gain  Gain=1/R(3)
  V2g_Micromega4 : Gain  Gain=1/R(4)
  V2g_Micromega5 : Gain  Gain=1/R(5)
  V2g_Micromega6 : Gain  Gain=1/R(6)
  acc1 : Outport  VectorParamsAs1DForOutWhenUnconnected=off
  acc2 : Outport  Port=2  VectorParamsAs1DForOutWhenUnconnected=off
  acc3 : Outport  Port=3  VectorParamsAs1DForOutWhenUnconnected=off
  acc4 : Outport  Port=4  VectorParamsAs1DForOutWhenUnconnected=off
  acc5 : Outport  Port=5  VectorParamsAs1DForOutWhenUnconnected=off
  acc6 : Outport  Port=6  VectorParamsAs1DForOutWhenUnconnected=off
  wires:
  V2g_Micromega2/1 -> Subsystem7/1(In1)
  Subsystem8/1(g2ms^2_Micromega3) -> acc3/1
  Subsystem11/1(g2ms^2_Micromega6) -> acc6/1
  V2g_Micromega4/1 -> Subsystem9/1(In1)
  V2g_Micromega1/1 -> Subsystem6/1(In1)
  Subsystem7/1(g2ms^2_Micromega2) -> acc2/1
  V2g_Micromega3/1 -> Subsystem8/1(In1)
  V2g_Micromega5/1 -> Subsystem10/1(In1)
  Subsystem9/1(g2ms^2_Micromega4) -> acc4/1
  Subsystem10/1(g2ms^2_Micromega5) -> acc5/1
  V2g_Micromega6/1 -> Subsystem11/1(In1)
  Subsystem6/1(g2ms^2_Micromega1) -> acc1/1
  GainADC_Ch18/1 -> V2g_Micromega2/1
  GainADC_Ch19/1 -> V2g_Micromega3/1
  GainADC_Ch17/1 -> V2g_Micromega1/1
  GainADC_Ch22/1 -> V2g_Micromega6/1
  GainADC_Ch21/1 -> V2g_Micromega5/1
  GainADC_Ch20/1 -> V2g_Micromega4/1

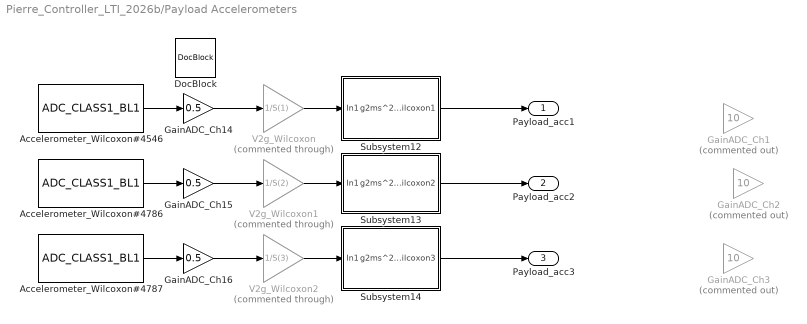
== system Pierre_Controller_LTI_2026b/Payload Accelerometers ==
  Accelerometer_Wilcoxon#4546 : rti1202lib_adc_class1/ADC_CLASS1_BL1  DSProperties=struct('RTI',struct('Version',uint32(1),'BlockType',struct('isSLSource',uint8(1),'isSLSink',uint8(1),'isHWSource',uint8(0),'isHWSink',uint8(1),'isSetup',uint8(0),'isInline',uint8(1),'isNonInline',uint8(0),'isInterrupt',uint8(0),'isChannelwise',uint8(1)),'IOBoardType',{{'DS120X','STD','ADCC1'}},'UnitType','ADC','Identifier','ADC','DialogType','ML','BlockSet','NONE','SlaveProcessor','NONE'))  RTIBlockInterface=struct('InputPortsActive',0,'InputPortsWidth',int32(1),'InputPortsDataType',{{'SS_BOOLEAN'}},'InputPortsName',{{'Continue'}},'OutputPortsActive',[1 0],'OutputPortsWidth',int32([1 1]),'OutputPortsDataType',{{'SS_DOUBLE','SS_INT16'}},'OutputPortsName',{{'ADC','Status'}},'DialogFcn','rti120xstdadcc1adcgui','SampleTime',{{-1}},'InitLevel',3,'IconTransparency','on','BlockDisplay',{{['ADC CL1\nChannel: 13'],'center'}},'BlockName',struct('Token',{{'ADC_CLASS1_BL1'}}))  RTIBlockParameters=struct('ReadMode',{{1,'OFF',[1 2]}},'ChannelNo',{{13,'OFF',[]}},'ConversionMode',{{1,'OFF',[1 2]}},'TriggerSource',{{1,'OFF',[1 2]}},'TriggerLineIn',{{1,'OFF',[1 16]}},'SampleMode',{{1,'OFF',[1 2]}},'BurstTriggerSource',{{1,'OFF',[1 2]}},'BurstTriggerLine',{{1,'OFF',[1 16]}},'ConvTriggerSource',{{3,'OFF',[1 3]}},'ConvTriggerLine',{{1,'OFF',[1 16]}},'ConvPeriod',{{'100e-6','OFF',[1e-6 1.34]}},'ConvPeriodCheck',{{0,'OFF',[]}},'BurstSize',{{'10','OFF',[]}},'BurstSizeCheck',{{0,'OFF',[]}},'DataSetOffset',{{'0','OFF',[]}},'DataSetOffsetCheck',{{0,'OFF',[]}},'DataSetLength',{{'1','OFF',[]}},'DataSetLengthCheck',{{0,'OFF',[]}},'EnableTriggerEvent',{{0,'OFF',[0 1]}},'TriggerMode',{{2,'OFF',[1 3]}},'TriggerLineOut',{{1,'OFF',[1 16]}},'ADCSWStartEnable',{{0,'OFF',[0 1]}},'SampleTime',{{'-1','OFF',[-1 inf]}},'SampleTimeCheck',{{1,'OFF',[]}},'StatusPortEnable',{{0,'OFF',[0 1]}},'TLCFileName',{{'rti120xadc_c1_adc','OFF',[]}})  RTISFcnParameters=struct('ReadMode','int16','ChannelNo','int16','ConversionMode','int16','TriggerSource','int16','TriggerLineIn','int16','SampleMode','int16','BurstTriggerSource','int16','BurstTriggerLine','int16','ConvTriggerSource','int16','ConvTriggerLine','int16','ConvPeriod','double','BurstSize','int16','DataSetOffset','int16','DataSetLength','int16','EnableTriggerEvent','int16','TriggerMode','int16','TriggerLineOut','int16','ADCSWStartEnable','int16','SampleTime','double','StatusPortEnable','int16','TLCFileName','char')  RTIBlockParaDefault=struct('ReadMode',1,'ChannelNo',1,'ConversionMode',1,'TriggerSource',1,'TriggerLineIn',1,'SampleMode',1,'BurstTriggerSource',1,'BurstTriggerLine',1,'ConvTriggerSource',3,'ConvTriggerLine',1,'ConvPeriod',0.0001,'ConvPeriodCheck',0,'BurstSize',10,'BurstSizeCheck',0,'DataSetOffset',0,'DataSetOffsetCheck',0,'DataSetLength',1,'DataSetLengthCheck',0,'EnableTriggerEvent',0,'TriggerMode',2,'TriggerLineOut',1,'ADCSWStartEnable',0,'SampleTime',-1,'SampleTimeCheck',1,'StatusPortEnable',0,'TLCFileName','rti120xadc_c1_adc')
  Accelerometer_Wilcoxon#4786 : rti1202lib_adc_class1/ADC_CLASS1_BL1  DSProperties=struct('RTI',struct('Version',uint32(1),'BlockType',struct('isSLSource',uint8(1),'isSLSink',uint8(1),'isHWSource',uint8(0),'isHWSink',uint8(1),'isSetup',uint8(0),'isInline',uint8(1),'isNonInline',uint8(0),'isInterrupt',uint8(0),'isChannelwise',uint8(1)),'IOBoardType',{{'DS120X','STD','ADCC1'}},'UnitType','ADC','Identifier','ADC','DialogType','ML','BlockSet','NONE','SlaveProcessor','NONE'))  RTIBlockInterface=struct('InputPortsActive',0,'InputPortsWidth',int32(1),'InputPortsDataType',{{'SS_BOOLEAN'}},'InputPortsName',{{'Continue'}},'OutputPortsActive',[1 0],'OutputPortsWidth',int32([1 1]),'OutputPortsDataType',{{'SS_DOUBLE','SS_INT16'}},'OutputPortsName',{{'ADC','Status'}},'DialogFcn','rti120xstdadcc1adcgui','SampleTime',{{-1}},'InitLevel',3,'IconTransparency','on','BlockDisplay',{{['ADC CL1\nChannel: 14'],'center'}},'BlockName',struct('Token',{{'ADC_CLASS1_BL1'}}))  RTIBlockParameters=struct('ReadMode',{{1,'OFF',[1 2]}},'ChannelNo',{{14,'OFF',[]}},'ConversionMode',{{1,'OFF',[1 2]}},'TriggerSource',{{1,'OFF',[1 2]}},'TriggerLineIn',{{1,'OFF',[1 16]}},'SampleMode',{{1,'OFF',[1 2]}},'BurstTriggerSource',{{1,'OFF',[1 2]}},'BurstTriggerLine',{{1,'OFF',[1 16]}},'ConvTriggerSource',{{3,'OFF',[1 3]}},'ConvTriggerLine',{{1,'OFF',[1 16]}},'ConvPeriod',{{'100e-6','OFF',[1e-6 1.34]}},'ConvPeriodCheck',{{0,'OFF',[]}},'BurstSize',{{'10','OFF',[]}},'BurstSizeCheck',{{0,'OFF',[]}},'DataSetOffset',{{'0','OFF',[]}},'DataSetOffsetCheck',{{0,'OFF',[]}},'DataSetLength',{{'1','OFF',[]}},'DataSetLengthCheck',{{0,'OFF',[]}},'EnableTriggerEvent',{{0,'OFF',[0 1]}},'TriggerMode',{{2,'OFF',[1 3]}},'TriggerLineOut',{{1,'OFF',[1 16]}},'ADCSWStartEnable',{{0,'OFF',[0 1]}},'SampleTime',{{'-1','OFF',[-1 inf]}},'SampleTimeCheck',{{1,'OFF',[]}},'StatusPortEnable',{{0,'OFF',[0 1]}},'TLCFileName',{{'rti120xadc_c1_adc','OFF',[]}})  RTISFcnParameters=struct('ReadMode','int16','ChannelNo','int16','ConversionMode','int16','TriggerSource','int16','TriggerLineIn','int16','SampleMode','int16','BurstTriggerSource','int16','BurstTriggerLine','int16','ConvTriggerSource','int16','ConvTriggerLine','int16','ConvPeriod','double','BurstSize','int16','DataSetOffset','int16','DataSetLength','int16','EnableTriggerEvent','int16','TriggerMode','int16','TriggerLineOut','int16','ADCSWStartEnable','int16','SampleTime','double','StatusPortEnable','int16','TLCFileName','char')  RTIBlockParaDefault=struct('ReadMode',1,'ChannelNo',1,'ConversionMode',1,'TriggerSource',1,'TriggerLineIn',1,'SampleMode',1,'BurstTriggerSource',1,'BurstTriggerLine',1,'ConvTriggerSource',3,'ConvTriggerLine',1,'ConvPeriod',0.0001,'ConvPeriodCheck',0,'BurstSize',10,'BurstSizeCheck',0,'DataSetOffset',0,'DataSetOffsetCheck',0,'DataSetLength',1,'DataSetLengthCheck',0,'EnableTriggerEvent',0,'TriggerMode',2,'TriggerLineOut',1,'ADCSWStartEnable',0,'SampleTime',-1,'SampleTimeCheck',1,'StatusPortEnable',0,'TLCFileName','rti120xadc_c1_adc')
  Accelerometer_Wilcoxon#4787 : rti1202lib_adc_class1/ADC_CLASS1_BL1  DSProperties=struct('RTI',struct('Version',uint32(1),'BlockType',struct('isSLSource',uint8(1),'isSLSink',uint8(1),'isHWSource',uint8(0),'isHWSink',uint8(1),'isSetup',uint8(0),'isInline',uint8(1),'isNonInline',uint8(0),'isInterrupt',uint8(0),'isChannelwise',uint8(1)),'IOBoardType',{{'DS120X','STD','ADCC1'}},'UnitType','ADC','Identifier','ADC','DialogType','ML','BlockSet','NONE','SlaveProcessor','NONE'))  RTIBlockInterface=struct('InputPortsActive',0,'InputPortsWidth',int32(1),'InputPortsDataType',{{'SS_BOOLEAN'}},'InputPortsName',{{'Continue'}},'OutputPortsActive',[1 0],'OutputPortsWidth',int32([1 1]),'OutputPortsDataType',{{'SS_DOUBLE','SS_INT16'}},'OutputPortsName',{{'ADC','Status'}},'DialogFcn','rti120xstdadcc1adcgui','SampleTime',{{-1}},'InitLevel',3,'IconTransparency','on','BlockDisplay',{{['ADC CL1\nChannel: 15'],'center'}},'BlockName',struct('Token',{{'ADC_CLASS1_BL1'}}))  RTIBlockParameters=struct('ReadMode',{{1,'OFF',[1 2]}},'ChannelNo',{{15,'OFF',[]}},'ConversionMode',{{1,'OFF',[1 2]}},'TriggerSource',{{1,'OFF',[1 2]}},'TriggerLineIn',{{1,'OFF',[1 16]}},'SampleMode',{{1,'OFF',[1 2]}},'BurstTriggerSource',{{1,'OFF',[1 2]}},'BurstTriggerLine',{{1,'OFF',[1 16]}},'ConvTriggerSource',{{3,'OFF',[1 3]}},'ConvTriggerLine',{{1,'OFF',[1 16]}},'ConvPeriod',{{'100e-6','OFF',[1e-6 1.34]}},'ConvPeriodCheck',{{0,'OFF',[]}},'BurstSize',{{'10','OFF',[]}},'BurstSizeCheck',{{0,'OFF',[]}},'DataSetOffset',{{'0','OFF',[]}},'DataSetOffsetCheck',{{0,'OFF',[]}},'DataSetLength',{{'1','OFF',[]}},'DataSetLengthCheck',{{0,'OFF',[]}},'EnableTriggerEvent',{{0,'OFF',[0 1]}},'TriggerMode',{{2,'OFF',[1 3]}},'TriggerLineOut',{{1,'OFF',[1 16]}},'ADCSWStartEnable',{{0,'OFF',[0 1]}},'SampleTime',{{'-1','OFF',[-1 inf]}},'SampleTimeCheck',{{1,'OFF',[]}},'StatusPortEnable',{{0,'OFF',[0 1]}},'TLCFileName',{{'rti120xadc_c1_adc','OFF',[]}})  RTISFcnParameters=struct('ReadMode','int16','ChannelNo','int16','ConversionMode','int16','TriggerSource','int16','TriggerLineIn','int16','SampleMode','int16','BurstTriggerSource','int16','BurstTriggerLine','int16','ConvTriggerSource','int16','ConvTriggerLine','int16','ConvPeriod','double','BurstSize','int16','DataSetOffset','int16','DataSetLength','int16','EnableTriggerEvent','int16','TriggerMode','int16','TriggerLineOut','int16','ADCSWStartEnable','int16','SampleTime','double','StatusPortEnable','int16','TLCFileName','char')  RTIBlockParaDefault=struct('ReadMode',1,'ChannelNo',1,'ConversionMode',1,'TriggerSource',1,'TriggerLineIn',1,'SampleMode',1,'BurstTriggerSource',1,'BurstTriggerLine',1,'ConvTriggerSource',3,'ConvTriggerLine',1,'ConvPeriod',0.0001,'ConvPeriodCheck',0,'BurstSize',10,'BurstSizeCheck',0,'DataSetOffset',0,'DataSetOffsetCheck',0,'DataSetLength',1,'DataSetLengthCheck',0,'EnableTriggerEvent',0,'TriggerMode',2,'TriggerLineOut',1,'ADCSWStartEnable',0,'SampleTime',-1,'SampleTimeCheck',1,'StatusPortEnable',0,'TLCFileName','rti120xadc_c1_adc')
  DocBlock : simulink/Model-Wide Utilities/DocBlock  DocumentType=Text
      content=|
      | Put the range of the charge amplifier here, typically 0.5 g. The dSpace DAQ
      | amplification factor of 10 is omitted as the voltage range of the charge
      | amplifier is also 10. Hence acceleration output = 0.5g * 10V (dSpace) / 10V
      | (amplifier).
  GainADC_Ch1 : Gain  Commented=on  Gain=10
  GainADC_Ch14 : Gain  Gain=0.5
  GainADC_Ch15 : Gain  Gain=0.5
  GainADC_Ch16 : Gain  Gain=0.5
  GainADC_Ch2 : Gain  Commented=on  Gain=10
  GainADC_Ch3 : Gain  Commented=on  Gain=10
  Subsystem12 : Subsystem
  Subsystem13 : Subsystem
  Subsystem14 : Subsystem
  V2g_Wilcoxon : Gain  Commented=through  Gain=1/S(1)
  V2g_Wilcoxon1 : Gain  Commented=through  Gain=1/S(2)
  V2g_Wilcoxon2 : Gain  Commented=through  Gain=1/S(3)
  Payload_acc1 : Outport  VectorParamsAs1DForOutWhenUnconnected=off
  Payload_acc2 : Outport  Port=2  VectorParamsAs1DForOutWhenUnconnected=off
  Payload_acc3 : Outport  Port=3  VectorParamsAs1DForOutWhenUnconnected=off
  wires:
  GainADC_Ch15/1 -> V2g_Wilcoxon1/1
  Accelerometer_Wilcoxon#4786/1 -> GainADC_Ch15/1
  GainADC_Ch14/1 -> V2g_Wilcoxon/1
  Accelerometer_Wilcoxon#4546/1 -> GainADC_Ch14/1
  GainADC_Ch16/1 -> V2g_Wilcoxon2/1
  Accelerometer_Wilcoxon#4787/1 -> GainADC_Ch16/1
  V2g_Wilcoxon/1 -> Subsystem12/1(In1)
  Subsystem12/1(g2ms^2_Wilcoxon1) -> Payload_acc1/1
  V2g_Wilcoxon2/1 -> Subsystem14/1(In1)
  Subsystem14/1(g2ms^2_Wilcoxon3) -> Payload_acc3/1
  V2g_Wilcoxon1/1 -> Subsystem13/1(In1)
  Subsystem13/1(g2ms^2_Wilcoxon2) -> Payload_acc2/1
